simulink model "prob4_lab3"  (R2025b)
settings: Solver=VariableStepAuto  StartTime=0.0  StopTime=10  RelTol=1e-3
libraries: dspsigops x3, simulink x1
settings Model: Creator=vivian.sleem  LastModifiedBy=vivian.sleem

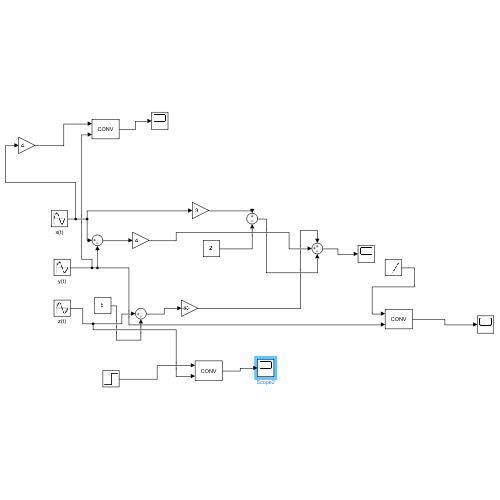
[thumbnail: Simulink's stored preview of the top-level diagram]
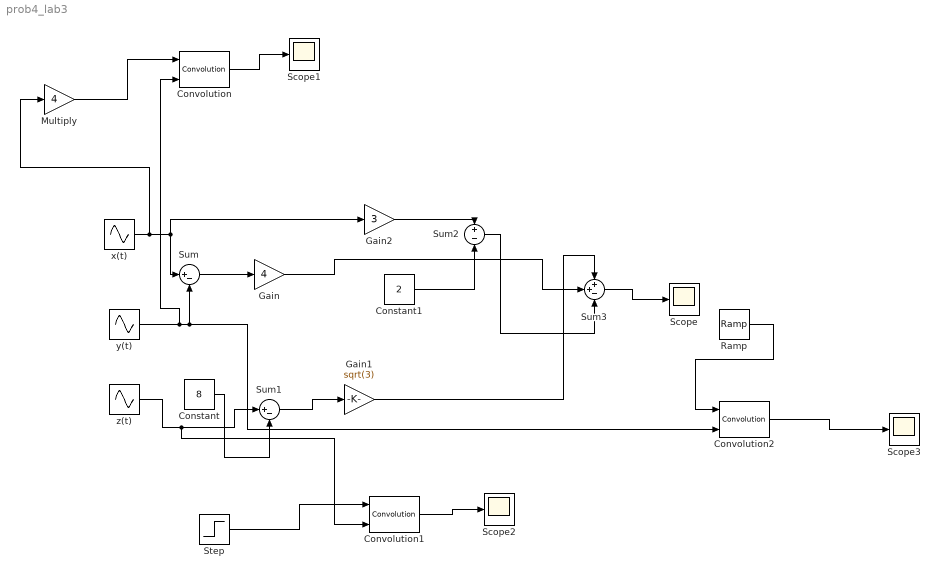
== system prob4_lab3 ==
  Constant : Constant  Value=8
  Constant1 : Constant  Value=2
  Convolution : dspsigops/Convolution  domain=Time  roundingMode=Floor  overflowMode=off  outputDataTypeStr=Inherit: Same as accumulator  outputMin=[]  outputMax=[]  outputLastDataTypeStr=Inherit: Same as accumulator
  Convolution1 : dspsigops/Convolution  domain=Time  roundingMode=Floor  overflowMode=off  outputDataTypeStr=Inherit: Same as accumulator  outputMin=[]  outputMax=[]  outputLastDataTypeStr=Inherit: Same as accumulator
  Convolution2 : dspsigops/Convolution  domain=Time  roundingMode=Floor  overflowMode=off  outputDataTypeStr=Inherit: Same as accumulator  outputMin=[]  outputMax=[]  outputLastDataTypeStr=Inherit: Same as accumulator
  Gain : Gain  Gain=4
  Gain1 : Gain  Gain=sqrt(3)
  Gain2 : Gain  Gain=3
  Multiply : Gain  Gain=4
  Ramp : simulink/Sources/Ramp  slope=1  start=0  InitialOutput=0
  Scope{,1..3} (4 alike) : Scope
      Scope settings: ActiveDisplayYMinimum=-1  ActiveDisplayYMaximum=1
      Scope1 settings: ActiveDisplayYMinimum=-1  ActiveDisplayYMaximum=1
      Scope2 settings: ActiveDisplayYMinimum=-2.6334932733619318  ActiveDisplayYMaximum=1.1750087137752656  DataLoggingVariableName=ScopeData2
      Scope3 settings: ActiveDisplayYMinimum=-104.55193126335369  ActiveDisplayYMaximum=124.7641572609069  DataLoggingVariableName=ScopeData3
  Step : Step  SampleTime=0
  Sum : Sum  Inputs=|+-
  Sum1 : Sum  Inputs=|+-
  Sum2 : Sum  Inputs=+-
  Sum3 : Sum  Inputs=++-
  x(t) : Sin  Frequency=5  SampleTime=0
  y(t) : Sin  Amplitude=0.5  SampleTime=0
  z(t) : Sin  Amplitude=2  Frequency=15  SampleTime=0
  wires:
  x(t)/1 -> Multiply/1, Gain2/1, Sum/1
  y(t)/1 -> Convolution2/2, Sum/2, Convolution/2
  Sum/1 -> Gain/1
  z(t)/1 -> Convolution1/2, Sum1/1
  Constant/1 -> Sum1/2
  Sum1/1 -> Gain1/1
  Constant1/1 -> Sum2/2
  Gain2/1 -> Sum2/1
  Gain/1 -> Sum3/2
  Gain1/1 -> Sum3/1
  Sum2/1 -> Sum3/3
  Sum3/1 -> Scope/1
  Multiply/1 -> Convolution/1
  Convolution/1 -> Scope1/1
  Step/1 -> Convolution1/1
  Convolution1/1 -> Scope2/1
  Ramp/1 -> Convolution2/1
  Convolution2/1 -> Scope3/1
